simulink model "NCO_FIR"  (R2026b)
settings: Solver=FixedStepAuto  StopTime=0.5
undefined symbols (not defined in the file): dspblkCoreblockFVToolHelper, gcbh
libraries: dspsrcs4 x1
settings Model: Creator=Gene  LastModifiedBy=Gene

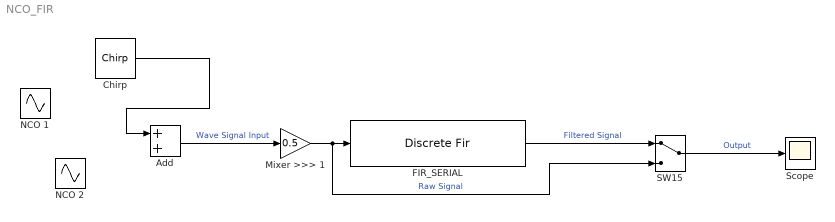
== system NCO_FIR ==
  Add : Sum
  Chirp : dspsrcs4/Chirp  SweepType=Linear  SweepDirection=Unidirectional  InitialFrequency=0  TargetFrequency=8000  TargetTime=0.5  SweepTime=1  InitialPhase=0  SampleTime=1/48828.125  SamplesPerFrame=1  OutputDataType=double  OutputFrames=off
  FIR_SERIAL : DiscreteFir  LoadFcn=dspblkCoreblockFVToolHelper(gcbh,'load');  Coefficients=fir1(62, 3000/(48828.125/2))
      settings: CopyFcn=dspblkCoreblockFVToolHelper(gcbh,'copy');  DeleteFcn=dspblkCoreblockFVToolHelper(gcbh,'close');  ModelCloseFcn=dspblkCoreblockFVToolHelper(gcbh,'close');  PreSaveFcn=dspblkCoreblockFVToolHelper(gcbh,'presave');  PostSaveFcn=dspblkCoreblockFVToolHelper(gcbh,'postsave');  CloseFcn=dspblkCoreblockFVToolHelper(gcbh,'close');
  Mixer >>> 1 : Gain  Gain=0.5
  NCO 1 : Sin  Frequency=1000*2*pi  SampleTime=1/48828.125
  NCO 2 : Sin  Frequency=8000*2*pi  SampleTime=1/48828.125
  SW15 : ManualSwitch
  Scope : Scope
      settings: ActiveDisplayYMinimum=-2.0918432451880742  ActiveDisplayYMaximum=2.7380436530596954
  wires:
  Add/1 -> Mixer >>> 1/1  "Wave Signal Input"
  Mixer >>> 1/1 -> SW15/2, FIR_SERIAL/1  "Raw Signal"
  FIR_SERIAL/1 -> SW15/1  "Filtered Signal"
  SW15/1 -> Scope/1  "Output"
  Chirp/1 -> Add/1
